simulink model "QEITest"  (Simulink 6.6)
settings: Solver=FixedStepDiscrete  StartTime=0.0  StopTime=10.0  FixedStep=0.001  RelTol=1e-3
undefined symbols (not defined in the file or in its folder): QEIInit
libraries: dsPICdrivers x9, simulink x2
settings Model: Creator=ASL_Lab  LastModifiedBy=ASL_Lab  ProdHWDeviceType=16-bit Generic
settings OptimizationCC: OptimizeModelRefInitCode=on  LifeSpan=1
settings HardwareCC: ProdBitPerInt=16  ProdEndianess=LittleEndian  ProdWordSize=16  ProdHWDeviceType=16-bit Generic  TargetHWDeviceType=32-bit Generic
settings RTWCC: SystemTargetFile=dspic.tlc  TemplateMakefile=dspic_pic30_gcc.tmf  PostCodeGenCommand=dsPIC_Compile()  Description=Embedded Target for Microchip dsPIC (real-time)  ProcessScript=dspic_make_rtw_hook  CustomSource=myQEI.c
settings CodeAppCC: IgnoreCustomStorageClasses=off
settings STFCustomTargetCC: TargetFcnLib=ansi_tfl_tmw.mat  GenFloatMathFcnCalls=ANSI_C  ModelReferenceCompliant=off  IncludeMdlTerminateFcn=off  CombineOutputUpdateFcns=on  SuppressErrorStatus=on  ERTCustomFileBanners=on  SupportContinuousTime=off  SupportNonInlinedSFcns=off  SystemTargetFile=dspic.tlc
settings ERTTargetCC: TargetFcnLib=ansi_tfl_tmw.mat  GenFloatMathFcnCalls=ANSI_C  ModelReferenceCompliant=off  IncludeMdlTerminateFcn=off  SuppressErrorStatus=on  ModelStepFunctionPrototypeControlCompliant=off  InlinedParameterPlacement=NonHierarchical  ERTSrcFileBannerTemplate=dsPIC_code_template.cgt  ERTHdrFileBannerTemplate=dsPIC_code_template.cgt  ERTDataSrcFileTemplate=dsPIC_code_template.cgt  ERTDataHdrFileTemplate=dsPIC_code_template.cgt  ERTCustomFileTemplate=dsPIC_main.tlc
settings CustomProperty: DataType=string  Value=C:\PROGRA~1\MATLAB\R2007a\rtw\bin\win32\gmake

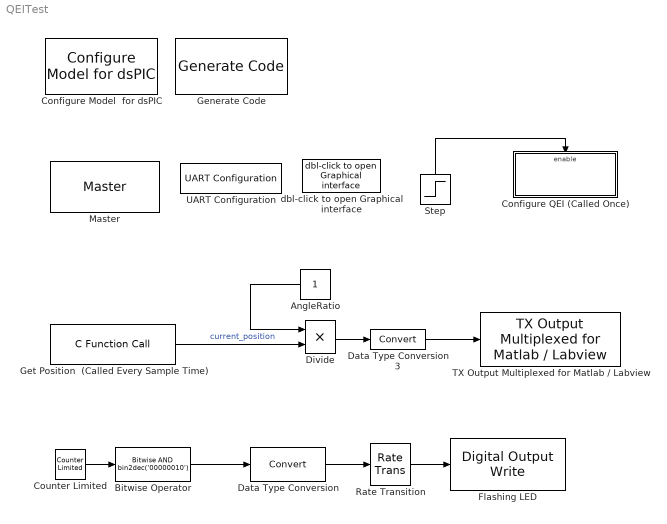
== system QEITest ==
  AngleRatio : Constant  Orientation=left  SampleTime=-1
  Bitwise Operator : simulink/Logic and Bit Operations/Bitwise Operator  logicop=AND  UseBitMask=on  BitMask=bin2dec('00000010')  BitMaskRealWorld=Stored Integer
  Configure Model  for dsPIC : dsPICdrivers/Simulink Configuration/Configure Model  for dsPIC
  Configure QEI (Called Once) : Subsystem  TreatAsAtomicUnit=on
  Counter Limited : simulink/Sources/Counter Limited  SystemSampleTime=-1  uplimit=3  tsamp=.25
  Data Type Conversion : DataTypeConversion  OutDataTypeMode=boolean
  Data Type Conversion3 : DataTypeConversion  OutDataTypeMode=int16
  Divide : Product  Inputs=**  OutScaling=2^-10
  Flashing LED : dsPICdrivers/Digital I//O/Digital Output Write  Tag=dsPIC_Digital_Output  Priority=5  PORT=D  Pin=[2]  Simultaneous=off  OrderingInOutPopup=None
  Generate Code : dsPICdrivers/Simulink Configuration/Generate Code
  Get Position  (Called Every Sample Time) : dsPICdrivers/OTHERS/C Function Call  Tag=dsPIC_dsPIC_CFunctionCall  fctName='GetQEI'  INPUT_SIZE=1  INPUT1=--  INPUT2=--  INPUT3=--  OUTPUT_SIZE=1  OUTPUT1=int32  SampleTime=-1  InputType=[ ]  OutputType=[ 5 ]  FctDeclaration=extern int32_T GetQEI();  FctCall=%y1 = GetQEI();  OrderingInOutPopup=None
  Master : dsPICdrivers/Master  Tag=dsPIC_MASTER  Priority=1  TimeStepType=Timer1  picType=30f4011  fcy=20e6  Quartz_33f=8e6  PLLActive_33f=off  fcyDesired_33f=4000000  tmr1="[1  19999  0]"  tmr1Info="Time Step : 0.001  ;   Error : 0%  PR1=19999"  tmr2345="[0  0  0  0]"  tmr2345cfg=[-1 -1 -1 -1]  IOautoConf=on  typePort="[ 0   0   0   0   0   0   0   0   0   0   0   0   0   0   0   0   0   0   0   0   0   0   0   0   0   0   0   0   0   0   0   0   0   0   0   0   0   0   0   0   0   0   0   0   0   0   0   0  10  10  10   0   0   0   0   0   0   0   0   0   0   0   0   0   0   0   0   0   0   0   0   0   0   0   0   0   0   0   0   0   0   0   0   0   4   5   0   0   0   0   0   0   0   0   0   0   0   0   0   0   0   0   0   0   0   0   0   0   0   0   0   0 ]"  TRIS="[ 65535  65535  65535  65528  65535  65535  65535 ]"  ADPCFG=0  MasterBusyPort=D0  MasterOverloadPort=D1  FOSC=XT_PLL8  TempProtection_33f=TEMP_ON  FPBOR=PBOR_OFF  PWRT=PWRT_OFF  MCLR=MCLR_EN  PowerSave=off
  Rate Transition : RateTransition  OutPortSampleTime=.001
  Step : Step  Orientation=up  Time=0.002  Before=1  After=0  SampleTime=0.001
  TX Output Multiplexed for Matlab / Labview : dsPICdrivers/Serial PORT/TX Output Multiplexed for Matlab // Labview  Tag=dsPIC_TX_Multiplexed  Priority=5  UART=2  CleverSpreadingChk=on  CleverSpreading=1  CHANNEL=[0]  BUFFERSIZE=128  CHANNELBLOCKED=[]  CHANNELBLOCKED_BITEWISE=0  Status=OK
  UART Configuration : dsPICdrivers/Serial PORT/UART Configuration  Tag=dsPIC_config_UART  Priority=2  UART=2  proposed_BAUD=19200  ALT_TX_RX=off  TXInterruptPri=7  InterruptTxWhen=When TxBUB has one empty space  TXEN=on  RXInterruptPri=1  BAUD=19200  UxBRG=64  Info="UxBRG = 64   ||  Real Baud : 19231   ||  % error : 0.16026  ||  max 1.9231 Bytes / Step"  RealBaud=0
  dbl-click to open Graphical interface : dsPICdrivers/Serial PORT/dbl-click to open Graphical interface  SystemSampleTime=-1
  wires:
  AngleRatio/1 -> Divide/1
  Divide/1 -> Data Type Conversion3/1
  Counter Limited/1 -> Bitwise Operator/1
  Bitwise Operator/1 -> Data Type Conversion/1
  Data Type Conversion/1 -> Rate Transition/1
  Rate Transition/1 -> Flashing LED/1
  Data Type Conversion3/1 -> TX Output Multiplexed for Matlab / Labview/1
  Step/1 -> Configure QEI (Called Once)/Enable
  Get Position  (Called Every Sample Time)/1 -> Divide/2  "current_position"

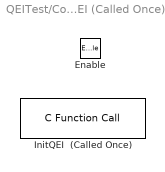
== system QEITest/Configure QEI (Called Once) ==
  Enable : EnablePort
  InitQEI  (Called Once) : dsPICdrivers/OTHERS/C Function Call  Tag=dsPIC_dsPIC_CFunctionCall  fctName='QEIInit'  INPUT_SIZE=1  INPUT1=--  INPUT2=--  INPUT3=--  OUTPUT_SIZE=1  OUTPUT1=--  SampleTime=inf  InputType=[ ]  OutputType=[ ]  FctDeclaration=extern void QEIInit();  FctCall=QEIInit();  OrderingInOutPopup=None
